simulink model "demoPanamaxContainerShip"  (R2022a)
settings: Solver=ode4  StartTime=0.0  StopTime=1500  FixedStep=0.5  RelTol=1e-6  AbsTol=1e-5  EnableMultiTasking=on
PreLoadFcn:
  | TT=40;
InitFcn:
  | dataPretoria;
StopFcn:
  | shipsOrient;
undefined symbols (not defined in the file): Ald, Are, c2, c3, Cayr, Cbyb, Cwmw, Cx0, D, Dp, Ir, Irm, Izz, k11, k22, k66, Kp, L, m1, m2, m3, m4, rho, Xe
libraries: simulink_extras x2, simulink x1
settings Model: Creator=Aleksander DP  LastModifiedBy=thor
settings SolverCC: AutoScaleAbsTol=off  AlgebraicLoopSolver=TrustRegion
settings DataIOCC: LimitDataPoints=on  SaveFormat=Array  SignalLoggingSaveFormat=ModelDataLogs  ReturnWorkspaceOutputs=off  SignalLoggingName=sigsOut
settings OptimizationCC: ExpressionDepthLimit=2147483647  InitFltsAndDblsToZero=on  LifeSpan=inf
settings DebuggingCC: SaveWithParameterizedLinksMsg=none  UnderspecifiedInitializationDetection=Classic  MergeDetectMultiDrivingBlocksExec=none  SignalResolutionControl=TryResolveAllWithWarning  MultiTaskDSMMsg=warning  MultiTaskCondExecSysMsg=none  FcnCallInpInsideContextMsg=warning  UnconnectedInputMsg=warning  UnconnectedOutputMsg=warning  UnconnectedLineMsg=warning  StateNameClashWarn=warning  SFUnexpectedBacktrackingDiag=warning  SFNoUnconditionalDefaultTransitionDiag=warning  SFExecutionAtInitializationDiag=none  SFMachineParentedDataDiag=warning  ArithmeticOperatorsInVariantConditions=warning
settings HardwareCC: ProdBitPerPointer=32  ProdBitPerSizeT=32  ProdBitPerPtrDiffT=32  ProdLargestAtomicFloat=None  ProdIntDivRoundTo=Undefined  ProdEndianess=Unspecified  ProdWordSize=32  ProdHWDeviceType=32-bit Generic  TargetUnknown=on
settings ModelReferenceCC: PropagateSignalLabelsOutOfModel=off
settings SFSimCC: SimUseLocalCustomCode=off  CustomCodeUndefinedFunction=UseInterfaceOnly
settings RTWCC: Description=Generic Real-Time Target  RTWUseLocalCustomCode=off  DLArmComputeVersion=19.05
settings CodeAppCC: StateflowObjectComments=on
settings GRTTargetCC: TargetFcnLib=ansi_tfl_tmw.mat  TargetLangStandard=C89/C90 (ANSI)  CombineOutputUpdateFcns=off  GRTInterface=on
settings ConfigComp: CovMetricSettings=dw  CovSaveCumulativeToWorkspaceVar=on  CovSaveSingleToWorkspaceVar=on  CovExternalEMLEnable=off

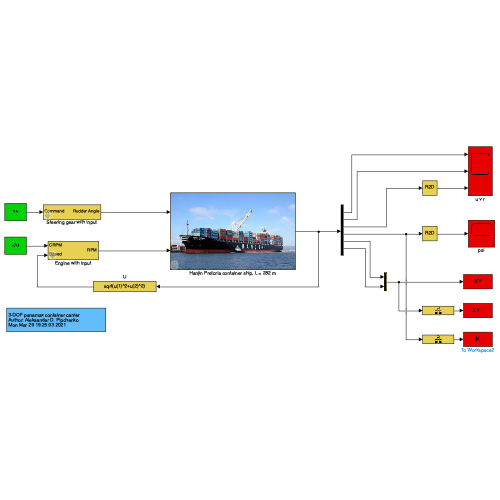
[thumbnail: Simulink's stored preview of the top-level diagram]
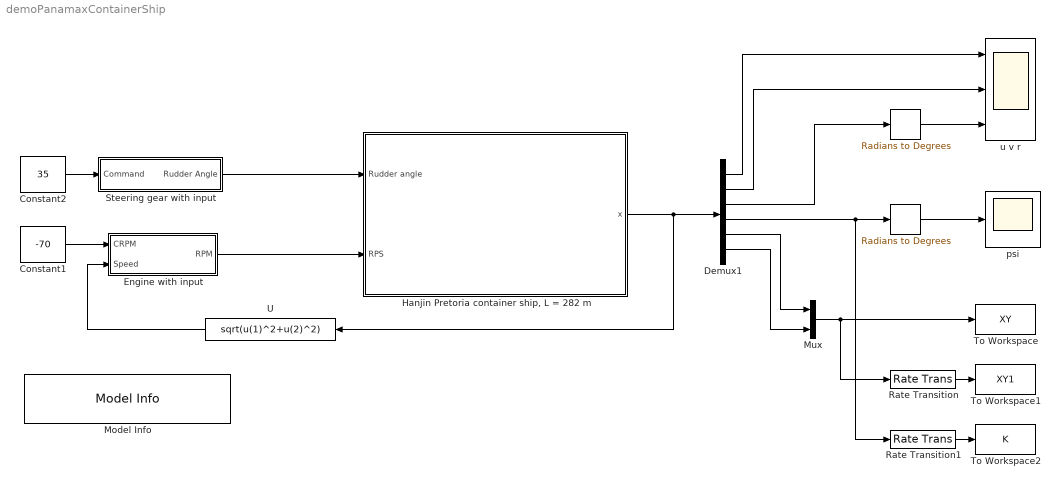
== system demoPanamaxContainerShip ==
  " " : simulink_extras/Transformations/Radians to Degrees
  "     " : simulink_extras/Transformations/Radians to Degrees
  Constant1 : Constant  Value=-70
  Constant2 : Constant  Value=35
  Demux1 : Demux  Outputs=6
  Engine with input : Subsystem  AncestorBlock=Maneuvering/Control complexes/Engine with input  mask(Engine (simplified)){IRPM=80, MaxRPM=100, MinRPM=-80, T_rpm=20, RevV=2.5, RTH=23, OTE=Revs per second}
      mask prompts: IRPM "Initial RPM, revs/min"; MaxRPM "Maximum RPM"; MinRPM "Minimum RPM"; T_rpm "Derrivative Time Constant"; RevV "Reversal speed, m/s"; RTH "RPM to keep ahead at crash stop, revs/min"; OTE "Output time expression"
      mask help:
      | Insert the reversal speed, and RPM ahead you want to hold
      | while ship not reach this speed at crash stop maneuver
      mask init:
      | if OTE=='Revs per minute'
      | 	TEX = 1;
      | elseif OTE=='Revs per second'
      | 	TEX = 1/60;
      | end;
      mask TypeOptions OTE: Revs per minute | Revs per second
  "Hanjin Pretoria container ship, L = 282 m" : Subsystem  mask(Ship 3-DOF model){IC=[10 0.001 0 0 0 0]}
      mask prompts: IC "Initial conditions [u v r psi X Y]"
      mask help:
      | Set ship's type in the model properties / init functions
      |
      | Inputs/outputs:
      |
      |    Rudder Angle     - set in radians
      |    RPS              - propeller revolutions per second
      |    x                - state vector [u v r psi X Y]
      mask Display: image('HanjinPretoria.jpg'); % Use "Edit Image" on toolstrip to change.
  Model Info : simulink/Model-Wide Utilities/Model Info  Frame=on  DisplayStringWithTags=|  HorizontalTextAlignment=Left  LeftAlignmentValue=0.02
      | 3-DOF panamax container carrier
      | Author: Aleksander D. Pipchenko
      | %<LastModificationDate>
  Mux : Mux  Inputs=2
  Rate Transition : RateTransition  OutPortSampleTime=TT
  Rate Transition1 : RateTransition  OutPortSampleTime=TT
  Steering gear with input : Subsystem  AncestorBlock=Maneuvering/Control complexes/Steering Gear with input  mask(Steering gear (simplified)){IRud=0, NSG=2, T_rud=20, DR=radians, MR=35, MRS=2.33, ST=-1}
      mask prompts: IRud "Intial Rudder angle, deg"; NSG "# of steering engnes in use"; T_rud "Derrivative time constant"; DR "Output values"; MR "Max. Rudder Angle, degrees"; MRS "Max. Rudder Speed, deg/second"; ST "Sample Time (-1 for inherited), s"
      mask init:
      | if DR=='degrees'
      | 	DRD = 1;
      | elseif DR=='radians'
      | 	DRD = pi/180;
      | end;
      mask TypeOptions NSG: 1 | 2
      mask TypeOptions DR: degrees | radians
  To Workspace : ToWorkspace  VariableName=XY  SampleTime=-1
  To Workspace1 : ToWorkspace  VariableName=XY1  SampleTime=TT
  To Workspace2 : ToWorkspace  VariableName=K  SampleTime=TT
  U : Fcn  Expr=sqrt(u(1)^2+u(2)^2)
  psi : Scope
  u v r : Scope  NumInputPorts=3
  wires:
  Constant2/1 -> Steering gear with input/1(Command)
  Constant1/1 -> Engine with input/1(CRPM)
  U/1 -> Engine with input/2(Speed)
  Steering gear with input/1(Rudder Angle) -> "Hanjin Pretoria container ship, L = 282 m"/1(Rudder angle)
  Engine with input/1(RPM) -> "Hanjin Pretoria container ship, L = 282 m"/2(RPS)
  "Hanjin Pretoria container ship, L = 282 m"/1(x) -> U/1, Demux1/1
  "     "/1 -> psi/1
  Rate Transition/1 -> To Workspace1/1
  Rate Transition1/1 -> To Workspace2/1
  " "/1 -> u v r/3
  Demux1/1 -> u v r/1
  Demux1/2 -> u v r/2
  Demux1/3 -> " "/1
  Mux/1 -> To Workspace/1, Rate Transition/1
  Demux1/4 -> "     "/1, Rate Transition1/1
  Demux1/5 -> Mux/1
  Demux1/6 -> Mux/2

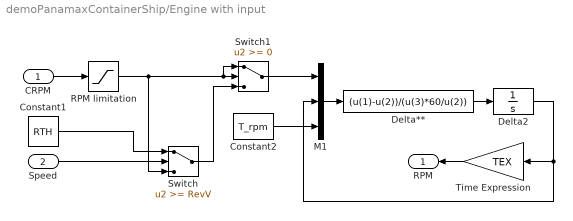
== system demoPanamaxContainerShip/Engine with input ==
  CRPM : Inport
  Speed : Inport  Port=2
  Constant1 : Constant  Value=RTH
  Constant2 : Constant  Value=T_rpm
  Delta** : Fcn  Expr=(u(1)-u(2))/(u(3)*60/u(2))
  Delta2 : Integrator  InitialCondition=IRPM  LimitOutput=on  UpperSaturationLimit=MaxRPM  LowerSaturationLimit=MinRPM
  M1 : Mux  Inputs=3
  RPM limitation : Saturate  UpperLimit=MaxRPM  LowerLimit=MinRPM
  Switch : Switch  Threshold=RevV  SaturateOnIntegerOverflow=off  InputSameDT=off
  Switch1 : Switch  SaturateOnIntegerOverflow=off  InputSameDT=off
  Time Expression : Gain  Gain=TEX
  RPM : Outport
  wires:
  Constant2/1 -> M1/3
  RPM limitation/1 -> Switch1/1, Switch1/2, Switch/3
  CRPM/1 -> RPM limitation/1
  Switch/1 -> Switch1/3
  Speed/1 -> Switch/2
  Switch1/1 -> M1/1
  Constant1/1 -> Switch/1
  M1/1 -> Delta**/1
  Delta**/1 -> Delta2/1
  Delta2/1 -> M1/2, Time Expression/1
  Time Expression/1 -> RPM/1

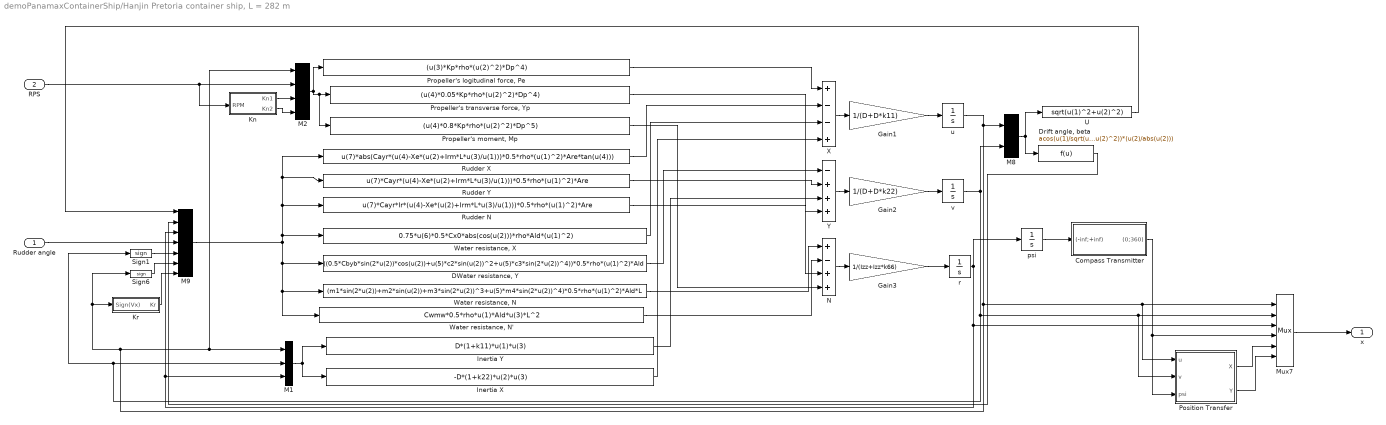
== system demoPanamaxContainerShip/Hanjin Pretoria container ship, L = 282 m ==
  Rudder angle : Inport
  RPS : Inport  Port=2
  Compass Transmitter : Subsystem  mask(Compass Transmitter){IVS=radians, OVS=radians}
      mask prompts: IVS "Input Value"; OVS "Output Value"
      mask help:
      | This block transfers the input value ranged (-inf;+inf) to value ranged (0;360) or (0;2*pi)
      | according to your choice.
      mask init:
      | if IVS =='degrees' 
      | 	IV =1;
      | elseif IVS =='radians'
      | 	IV = 180/pi;
      | end;
      | if OVS =='degrees'
      | 	OV =1;
      | elseif OVS=='radians'
      | 	OV=pi/180;
      | end;
      mask TypeOptions IVS: degrees | radians
      mask TypeOptions OVS: degrees | radians
  "DWater resistance, Y" : Fcn  Expr=((0.5*Cbyb*sin(2*u(2))*cos(u(2))+u(5)*c2*sin(u(2))^2+u(5)*c3*sin(2*u(2))^4))*0.5*rho*(u(1)^2)*Ald
  "Drift angle, beta" : Fcn  Expr=acos(u(1)/sqrt(u(1)^2+u(2)^2))*(u(2)/abs(u(2)))
  Gain1 : Gain  Gain=1/(D+D*k11)
  Gain2 : Gain  Gain=1/(D+D*k22)
  Gain3 : Gain  Gain=1/(Izz+Izz*k66)
  Inertia X : Fcn  Expr=-D*(1+k22)*u(2)*u(3)
  Inertia Y : Fcn  Expr=D*(1+k11)*u(1)*u(3)
  Kn : Subsystem
  Kr : Subsystem
  M1 : Mux  Inputs=3
  M2 : Mux
  M8 : Mux  Inputs=2
  M9 : Mux  Inputs=7
  Mux7 : Mux  Inputs=6
  N : Sum  Inputs=+-++  InputSameDT=on  SaturateOnIntegerOverflow=on  OutDataTypeStr=Inherit: Same as first input
  Position Transfer : Subsystem  mask(Position transfer, 2-D){CC=Meters, XY=[IC(5) IC(6)]}
      mask prompts: CC "XY dimension"; XY "Initial position"
      mask init:
      | if CC=='Cables'
      | 	MC = 1/185.23;
      | elseif CC=='Meters'
      | 	MC = 1;
      | end;
      | Xin = XY(1);Yin=XY(2);
      mask TypeOptions CC: Cables | Meters
  "Propeller's logitudinal force, Pe" : Fcn  Expr=(u(3)*Kp*rho*(u(2)^2)*Dp^4)
  "Propeller's moment, Mp" : Fcn  Expr=(u(4)*0.8*Kp*rho*(u(2)^2)*Dp^5)
  "Propeller's transverse force, Yp" : Fcn  Expr=(u(4)*0.05*Kp*rho*(u(2)^2)*Dp^4)
  Rudder N : Fcn  Expr=u(7)*Cayr*Ir*(u(4)-Xe*(u(2)+Irm*L*u(3)/u(1)))*0.5*rho*(u(1)^2)*Are
  Rudder X : Fcn  Expr=u(7)*abs(Cayr*(u(4)-Xe*(u(2)+Irm*L*u(3)/u(1)))*0.5*rho*(u(1)^2)*Are*tan(u(4)))
  Rudder Y : Fcn  Expr=u(7)*Cayr*(u(4)-Xe*(u(2)+Irm*L*u(3)/u(1)))*0.5*rho*(u(1)^2)*Are
  Sign1 : Signum
  Sign6 : Signum
  U : Fcn  Expr=sqrt(u(1)^2+u(2)^2)
  "Water resistance, N" : Fcn  Expr=(m1*sin(2*u(2))+m2*sin(u(2))+m3*sin(2*u(2))^3+u(5)*m4*sin(2*u(2))^4)*0.5*rho*(u(1)^2)*Ald*L
  "Water resistance, N'" : Fcn  Expr=Cwmw*0.5*rho*u(1)*Ald*u(3)*L^2
  "Water resistance, X" : Fcn  Expr=0.75*u(6)*0.5*Cx0*abs(cos(u(2)))*rho*Ald*(u(1)^2)
  X : Sum  Inputs=+--+  InputSameDT=on  SaturateOnIntegerOverflow=on  OutDataTypeStr=Inherit: Same as first input
  Y : Sum  Inputs=-+++  InputSameDT=on  SaturateOnIntegerOverflow=on  OutDataTypeStr=Inherit: Same as first input
  psi : Integrator  InitialCondition=IC(4)  UpperSaturationLimit=0.87266  LowerSaturationLimit=-0.87266  AbsoluteTolerance=1
  r : Integrator  InitialCondition=IC(3)  UpperSaturationLimit=0.87266  LowerSaturationLimit=-0.87266  AbsoluteTolerance=1
  u : Integrator  InitialCondition=IC(1)  UpperSaturationLimit=7.5  LowerSaturationLimit=-1  AbsoluteTolerance=1
  v : Integrator  InitialCondition=IC(2)  UpperSaturationLimit=7.5  LowerSaturationLimit=-1  AbsoluteTolerance=1
  x : Outport
  wires:
  M2/1 -> "Propeller's moment, Mp"/1, "Propeller's transverse force, Yp"/1, "Propeller's logitudinal force, Pe"/1
  M9/1 -> Rudder X/1, Rudder Y/1, Rudder N/1, "Water resistance, X"/1, "Water resistance, N"/1, "Water resistance, N'"/1, "DWater resistance, Y"/1
  "Propeller's logitudinal force, Pe"/1 -> X/1
  Rudder X/1 -> X/2
  Rudder Y/1 -> Y/2
  "Water resistance, X"/1 -> X/3
  "DWater resistance, Y"/1 -> Y/1
  "Water resistance, N"/1 -> N/1
  "Water resistance, N'"/1 -> N/2
  Rudder N/1 -> N/3
  U/1 -> M9/1
  v/1 -> M8/2, Sign1/1, M1/2, Mux7/2, Position Transfer/2(v)
  r/1 -> psi/1, M9/3, M1/3, Mux7/3
  u/1 -> M8/1, M1/1, M2/1, Sign6/1, Kr/1(Sign(Vx)), Mux7/1, Position Transfer/1(u)
  "Drift angle, beta"/1 -> M9/2
  Sign1/1 -> M9/5
  Sign6/1 -> M9/6
  Compass Transmitter/1((0;360)) -> Mux7/4, Position Transfer/3(psi)
  M1/1 -> Inertia X/1, Inertia Y/1
  X/1 -> Gain1/1
  Inertia X/1 -> X/4
  Gain1/1 -> u/1
  Y/1 -> Gain2/1
  Gain2/1 -> v/1
  Inertia Y/1 -> Y/3
  N/1 -> Gain3/1
  Gain3/1 -> r/1
  M8/1 -> U/1, "Drift angle, beta"/1
  psi/1 -> Compass Transmitter/1((-inf;+inf))
  "Propeller's transverse force, Yp"/1 -> Y/4
  "Propeller's moment, Mp"/1 -> N/4
  Kn/1(Kn1) -> M2/3
  Kn/2(Kn2) -> M2/4
  Kr/1(Kr) -> M9/7
  RPS/1 -> M2/2, Kn/1(RPM)
  Rudder angle/1 -> M9/4
  Mux7/1 -> x/1
  Position Transfer/1(X) -> Mux7/5
  Position Transfer/2(Y) -> Mux7/6

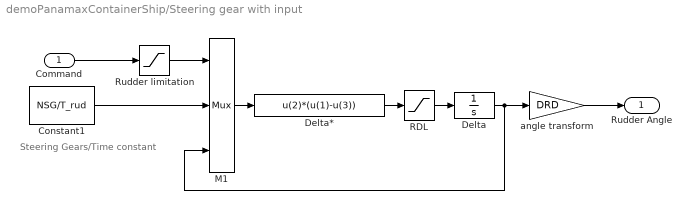
== system demoPanamaxContainerShip/Steering gear with input ==
  note: Steering Gears/Time constant
  Command : Inport
  Constant1 : Constant  Value=NSG/T_rud
  Delta : Integrator  InitialCondition=IRud  LimitOutput=on  UpperSaturationLimit=MR  LowerSaturationLimit=-MR
  Delta* : Fcn  Expr=u(2)*(u(1)-u(3))  SampleTime=ST
  M1 : Mux  Inputs=3
  RDL : Saturate  UpperLimit=MRS  LowerLimit=-MRS  SampleTime=ST
  Rudder limitation : Saturate  UpperLimit=MR  LowerLimit=-MR  SampleTime=ST
  angle transform : Gain  Gain=DRD  SampleTime=ST
  Rudder Angle : Outport
  wires:
  RDL/1 -> Delta/1
  angle transform/1 -> Rudder Angle/1
  Constant1/1 -> M1/2
  Rudder limitation/1 -> M1/1
  Delta/1 -> M1/3, angle transform/1
  Delta*/1 -> RDL/1
  M1/1 -> Delta*/1
  Command/1 -> Rudder limitation/1

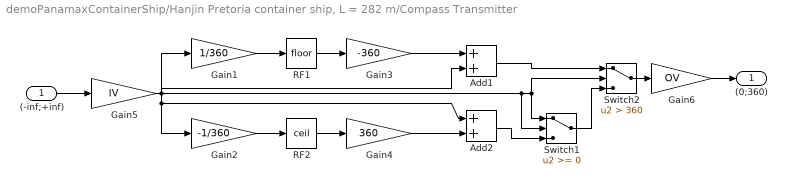
== system demoPanamaxContainerShip/Hanjin Pretoria container ship, L = 282 m/Compass Transmitter ==
  (-inf;+inf) : Inport
  Add1 : Sum
  Add2 : Sum
  Gain1 : Gain  Gain=1/360
  Gain2 : Gain  Gain=-1/360
  Gain3 : Gain  Gain=-360
  Gain4 : Gain  Gain=360
  Gain5 : Gain  Gain=IV
  Gain6 : Gain  Gain=OV
  RF1 : Rounding
  RF2 : Rounding  Operator=ceil
  Switch1 : Switch  SaturateOnIntegerOverflow=off  InputSameDT=off
  Switch2 : Switch  Criteria=u2 > Threshold  Threshold=360  SaturateOnIntegerOverflow=off  InputSameDT=off
  (0;360) : Outport
  wires:
  Gain6/1 -> (0;360)/1
  Gain5/1 -> Switch1/2, Switch2/2, Switch1/1, Gain1/1, Add1/2, Gain2/1, Add2/1
  Switch2/1 -> Gain6/1
  Switch1/1 -> Switch2/3
  Add2/1 -> Switch1/3
  Add1/1 -> Switch2/1
  Gain4/1 -> Add2/2
  Gain3/1 -> Add1/1
  RF2/1 -> Gain4/1
  RF1/1 -> Gain3/1
  Gain2/1 -> RF2/1
  Gain1/1 -> RF1/1
  (-inf;+inf)/1 -> Gain5/1

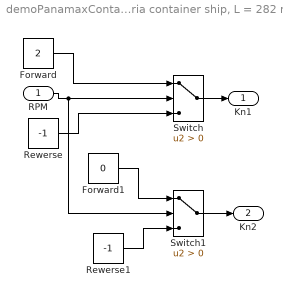
== system demoPanamaxContainerShip/Hanjin Pretoria container ship, L = 282 m/Kn ==
  RPM : Inport
  Forward : Constant  Value=2
  Forward1 : Constant  Value=0
  Rewerse : Constant  Value=-1
  Rewerse1 : Constant  Value=-1
  Switch : Switch  Criteria=u2 > Threshold  SaturateOnIntegerOverflow=off  InputSameDT=off
  Switch1 : Switch  Criteria=u2 > Threshold  SaturateOnIntegerOverflow=off  InputSameDT=off
  Kn1 : Outport
  Kn2 : Outport  Port=2
  wires:
  Forward/1 -> Switch/1
  Rewerse/1 -> Switch/3
  RPM/1 -> Switch/2, Switch1/2
  Switch/1 -> Kn1/1
  Forward1/1 -> Switch1/1
  Rewerse1/1 -> Switch1/3
  Switch1/1 -> Kn2/1

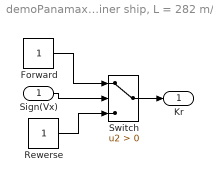
== system demoPanamaxContainerShip/Hanjin Pretoria container ship, L = 282 m/Kr ==
  Sign(Vx) : Inport
  Forward : Constant
  Rewerse : Constant
  Switch : Switch  Criteria=u2 > Threshold  SaturateOnIntegerOverflow=off  InputSameDT=off
  Kr : Outport
  wires:
  Forward/1 -> Switch/1
  Rewerse/1 -> Switch/3
  Sign(Vx)/1 -> Switch/2
  Switch/1 -> Kr/1

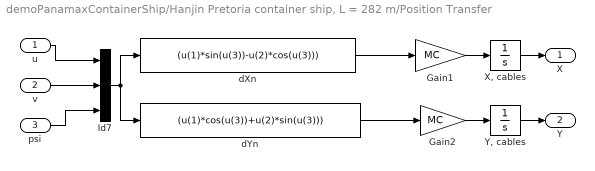
== system demoPanamaxContainerShip/Hanjin Pretoria container ship, L = 282 m/Position Transfer ==
  u : Inport
  v : Inport  Port=2
  psi : Inport  Port=3
  Gain1 : Gain  Gain=MC
  Gain2 : Gain  Gain=MC
  Id7 : Mux  Inputs=3
  "X, cables" : Integrator  InitialCondition=Xin
  "Y, cables" : Integrator  InitialCondition=Yin
  dXn : Fcn  Expr=(u(1)*sin(u(3))-u(2)*cos(u(3)))
  dYn : Fcn  Expr=(u(1)*cos(u(3))+u(2)*sin(u(3)))
  X : Outport
  Y : Outport  Port=2
  wires:
  v/1 -> Id7/2
  u/1 -> Id7/1
  Id7/1 -> dYn/1, dXn/1
  dXn/1 -> Gain1/1
  dYn/1 -> Gain2/1
  "X, cables"/1 -> X/1
  "Y, cables"/1 -> Y/1
  Gain1/1 -> "X, cables"/1
  Gain2/1 -> "Y, cables"/1
  psi/1 -> Id7/3
